simulink model "Sensor_Fusion_Simulink"  (R2025b)
settings: Solver=VariableStepAuto  StartTime=0.0  StopTime=30  RelTol=1e-3
undefined symbols (not defined in the file): DiscIntNeverNeededParam
libraries: simulink_extras x10, slpidlib x7, simulink x5
settings Model: Creator=Admin ROG  LastModifiedBy=Admin ROG

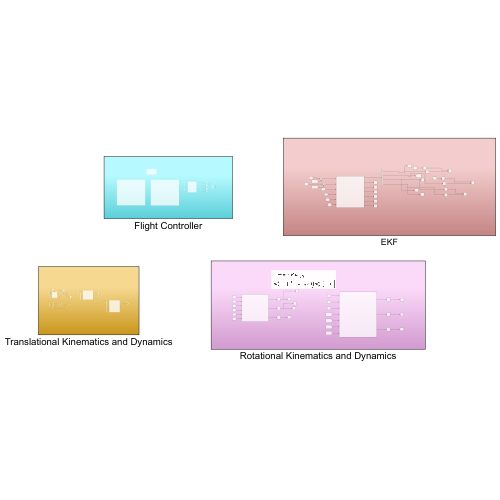
[thumbnail: Simulink's stored preview of the top-level diagram]
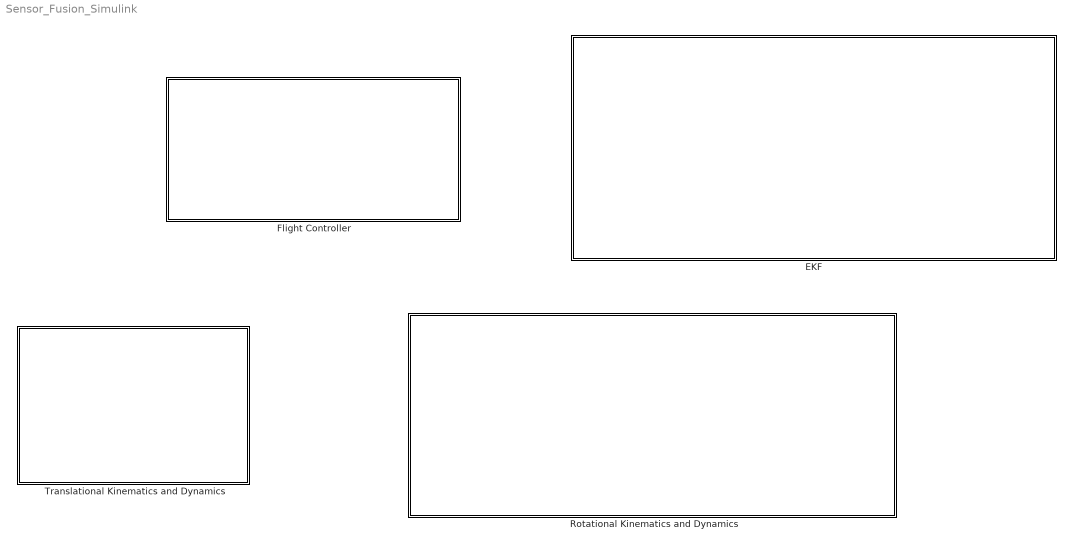
== system Sensor_Fusion_Simulink ==
  EKF : Subsystem
  Flight Controller : Subsystem
  Rotational Kinematics and Dynamics : Subsystem
  Translational Kinematics and Dynamics : Subsystem

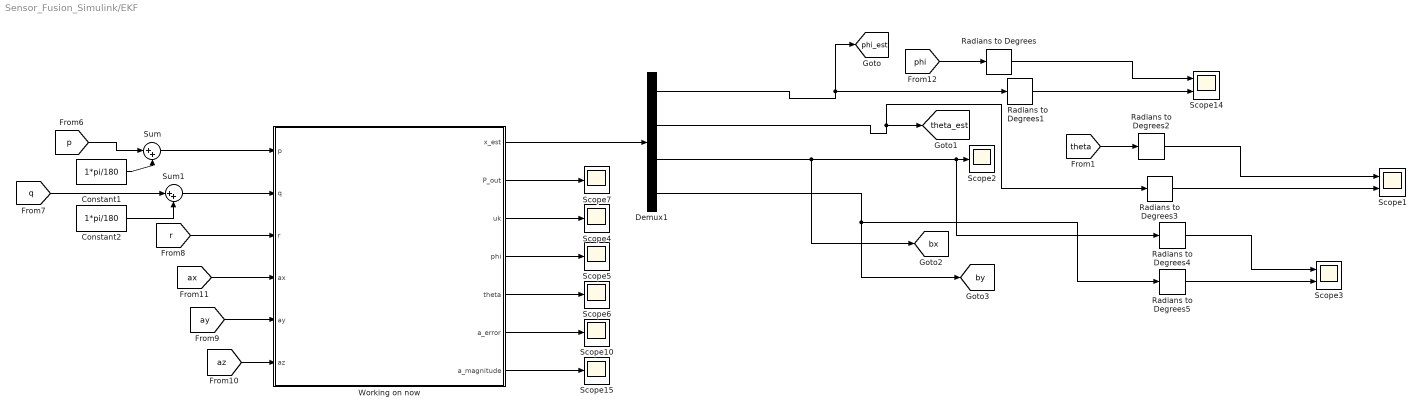
== system Sensor_Fusion_Simulink/EKF ==
  Constant1 : Constant  Value=1*pi/180
  Constant2 : Constant  Value=1*pi/180
  Demux1 : Demux
  Radians to Degrees{,1..5} (6 alike) : simulink_extras/Transformations/Radians to Degrees
  Scope1 : Scope  NumInputPorts=2
      settings: ActiveDisplayYMinimum=-0.57990177915773911  ActiveDisplayYMaximum=0.85703606877575134  DataLoggingVariableName=ScopeData19
  Scope{2,4..7,10,15} (7 alike) : Scope
      Scope10 settings: ActiveDisplayYMinimum=-33.495641453039809  ActiveDisplayYMaximum=182.18044745290689  DataLoggingVariableName=ScopeData35
      Scope15 settings: ActiveDisplayYMinimum=-33.295659158076418  ActiveDisplayYMaximum=317.12667362775773  DataLoggingVariableName=ScopeData36
      Scope2 settings: ActiveDisplayYMinimum=-0.0058388321761880082  ActiveDisplayYMaximum=0.025479521819259585  DataLoggingVariableName=ScopeData20
      Scope4 settings: ActiveDisplayYMinimum=-0.41125597879318471  ActiveDisplayYMaximum=3.5363536127434574  DataLoggingVariableName=ScopeData22
      Scope5 settings: ActiveDisplayYMinimum=-115.87931452635893  ActiveDisplayYMaximum=917.93819898150412  DataLoggingVariableName=ScopeData23
      Scope6 settings: ActiveDisplayYMinimum=-0.0043204427587799  ActiveDisplayYMaximum=0.014186886760105504  DataLoggingVariableName=ScopeData24
      Scope7 settings: ActiveDisplayYMinimum=-4.3708616172804561E-5  ActiveDisplayYMaximum=0.00012450012296327597  DataLoggingVariableName=ScopeData25
  Scope14 : Scope  NumInputPorts=2
      settings: ActiveDisplayYMinimum=-4.8648496704127089  ActiveDisplayYMaximum=36.951521266621747  DataLoggingVariableName=ScopeData18
  Scope3 : Scope  NumInputPorts=2
      settings: ActiveDisplayYMinimum=-0.33454044098075875  ActiveDisplayYMaximum=1.4598690642550676  DataLoggingVariableName=ScopeData21
  Sum : Sum  Inputs=|++
  Sum1 : Sum  Inputs=|++
  Working on now : MATLAB Function  TreatAsAtomicUnit=on
  tag scope: bx=global, by=global, phi_est=global, theta_est=global
  wires:
  Demux1/3 -> [bx], Radians to Degrees4/1, Scope2/1
  Sum/1 -> Working on now/1(p)
  Demux1/1 -> [phi_est], Radians to Degrees1/1
  [az] -> Working on now/6(az)
  [ax] -> Working on now/4(ax)
  [p] -> Sum/1
  Working on now/5(theta) -> Scope6/1
  Working on now/6(a_error) -> Scope10/1
  Demux1/4 -> [by], Radians to Degrees5/1
  Working on now/7(a_magnitude) -> Scope15/1
  Working on now/4(phi) -> Scope5/1
  [ay] -> Working on now/5(ay)
  Working on now/3(uk) -> Scope4/1
  Demux1/2 -> [theta_est], Radians to Degrees3/1
  Working on now/1(x_est) -> Demux1/1
  Working on now/2(P_out) -> Scope7/1
  [r] -> Working on now/3(r)
  [phi] -> Radians to Degrees/1
  Radians to Degrees/1 -> Scope14/1
  Radians to Degrees1/1 -> Scope14/2
  Constant1/1 -> Sum/2
  [q] -> Sum1/1
  Sum1/1 -> Working on now/2(q)
  Constant2/1 -> Sum1/2
  [theta] -> Radians to Degrees2/1
  Radians to Degrees2/1 -> Scope1/1
  Radians to Degrees3/1 -> Scope1/2
  Radians to Degrees4/1 -> Scope3/1
  Radians to Degrees5/1 -> Scope3/2

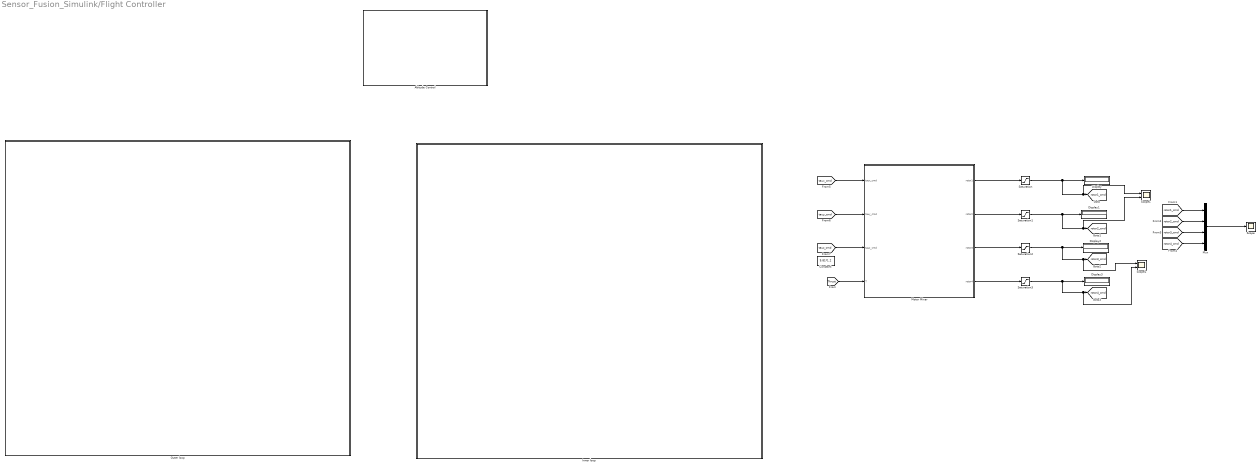
== system Sensor_Fusion_Simulink/Flight Controller ==
  Altitude Control : Subsystem
  Constant : Constant  Value=9.81*1.2
  Display{,1..3} (4 alike) : Display
  Inner loop : Subsystem
  Motor Mixer : MATLAB Function  TreatAsAtomicUnit=on
  Mux : Mux
  Outer loop : Subsystem
  Saturation{,1..3} (4 alike) : Saturate  UpperLimit=2094.8  LowerLimit=0
  Scope : Scope
      settings: ActiveDisplayYMinimum=-261.84999999999997  ActiveDisplayYMaximum=2356.65  DataLoggingVariableName=ScopeData7
  Scope1 : Scope  NumInputPorts=2
      settings: ActiveDisplayYMinimum=-261.84999999999997  ActiveDisplayYMaximum=2356.65  DataLoggingVariableName=ScopeData11
  Scope2 : Scope  NumInputPorts=2
      settings: ActiveDisplayYMinimum=820.27707495183745  ActiveDisplayYMaximum=820.27707495183768  DataLoggingVariableName=ScopeData12
  tag scope: rotor1_cmd=global, rotor2_cmd=global, rotor3_cmd=global, rotor4_cmd=global
  wires:
  [rotor2_cmd] -> Mux/2
  [rotor3_cmd] -> Mux/3
  Mux/1 -> Scope/1
  [rotor1_cmd] -> Mux/1
  [rotor4_cmd] -> Mux/4
  Motor Mixer/4(rotor4) -> Saturation3/1
  Motor Mixer/3(rotor3) -> Saturation2/1
  Motor Mixer/1(rotor1) -> Saturation/1
  Motor Mixer/2(rotor2) -> Saturation1/1
  Saturation/1 -> Scope1/1, [rotor1_cmd], Display/1
  Saturation1/1 -> Scope1/2, [rotor2_cmd], Display1/1
  Saturation2/1 -> Scope2/1, [rotor3_cmd], Display2/1
  Saturation3/1 -> Scope2/2, [rotor4_cmd], Display3/1
  [tauy_cmd] -> Motor Mixer/2(tauy_cmd)
  [taux_cmd] -> Motor Mixer/1(taux_cmd)
  [tauz_cmd] -> Motor Mixer/3(tauz_cmd)
  [Thrust] -> Motor Mixer/4(T)

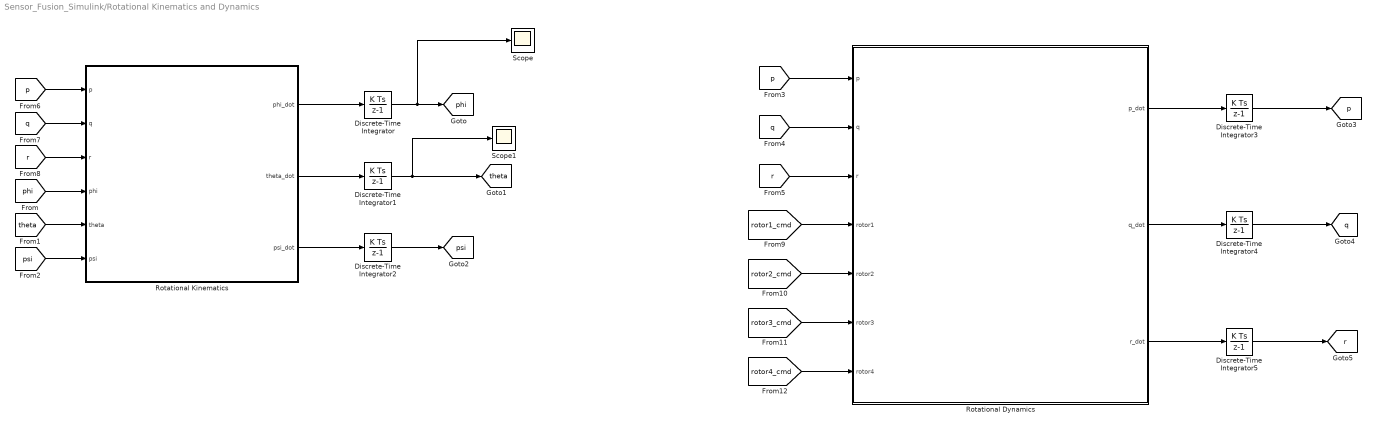
== system Sensor_Fusion_Simulink/Rotational Kinematics and Dynamics ==
  Discrete-Time Integrator{,1..5} (6 alike) : DiscreteIntegrator  SampleTime=0.002  ICPrevOutput=DiscIntNeverNeededParam  ICPrevScaledInput=DiscIntNeverNeededParam
  Rotational Dynamics : MATLAB Function  TreatAsAtomicUnit=on
  "Rotational Kinematics    " : MATLAB Function  TreatAsAtomicUnit=on
  Scope : Scope
      settings: ActiveDisplayYMinimum=-0.022412150722965766  ActiveDisplayYMaximum=0.028745169300771516  DataLoggingVariableName=ScopeData3
  Scope1 : Scope
      settings: ActiveDisplayYMinimum=-13.839906623900923  ActiveDisplayYMaximum=45.902212590490322  DataLoggingVariableName=ScopeData4
  tag scope: p=global, phi=global, psi=global, q=global, r=global, theta=global
  wires:
  Discrete-Time Integrator2/1 -> [psi]
  Discrete-Time Integrator4/1 -> [q]
  Discrete-Time Integrator/1 -> Scope/1, [phi]
  [psi] -> "Rotational Kinematics    "/6(psi)
  [theta] -> "Rotational Kinematics    "/5(theta)
  Discrete-Time Integrator3/1 -> [p]
  "Rotational Kinematics    "/1(phi_dot) -> Discrete-Time Integrator/1
  "Rotational Kinematics    "/2(theta_dot) -> Discrete-Time Integrator1/1
  "Rotational Kinematics    "/3(psi_dot) -> Discrete-Time Integrator2/1
  [phi] -> "Rotational Kinematics    "/4(phi)
  Rotational Dynamics/2(q_dot) -> Discrete-Time Integrator4/1
  Discrete-Time Integrator5/1 -> [r]
  Rotational Dynamics/3(r_dot) -> Discrete-Time Integrator5/1
  Rotational Dynamics/1(p_dot) -> Discrete-Time Integrator3/1
  [r] -> Rotational Dynamics/3(r)
  [q] -> Rotational Dynamics/2(q)
  [p] -> Rotational Dynamics/1(p)
  [p] -> "Rotational Kinematics    "/1(p)
  [q] -> "Rotational Kinematics    "/2(q)
  [r] -> "Rotational Kinematics    "/3(r)
  Discrete-Time Integrator1/1 -> Scope1/1, [theta]
  [rotor2_cmd] -> Rotational Dynamics/5(rotor2)
  [rotor1_cmd] -> Rotational Dynamics/4(rotor1)
  [rotor4_cmd] -> Rotational Dynamics/7(rotor4)
  [rotor3_cmd] -> Rotational Dynamics/6(rotor3)

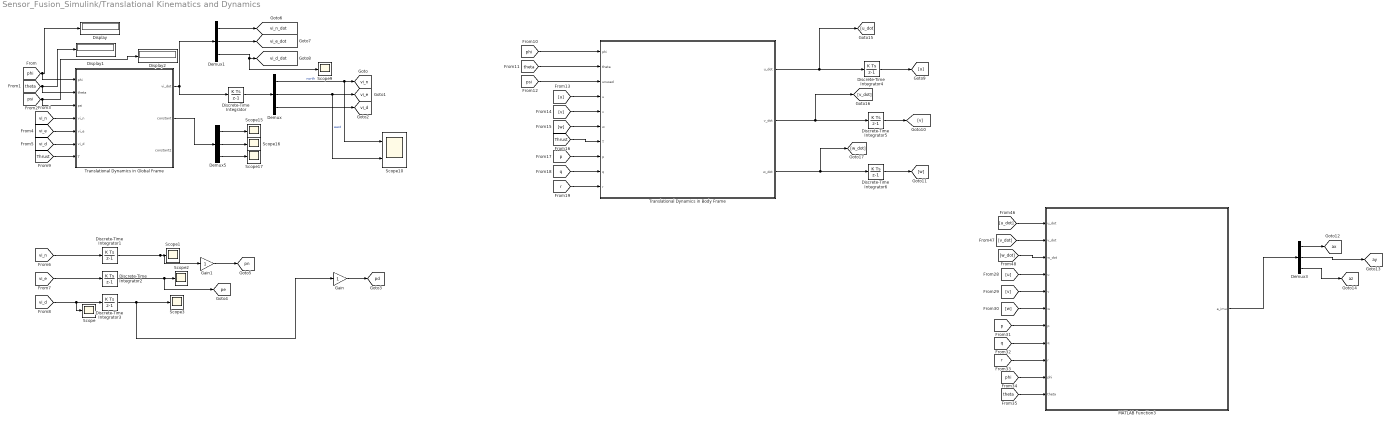
== system Sensor_Fusion_Simulink/Translational Kinematics and Dynamics ==
  Demux{,1,3,5} (4 alike) : Demux  Outputs=3
  Discrete-Time Integrator{,1..6} (7 alike) : DiscreteIntegrator  SampleTime=0.002  ICPrevOutput=DiscIntNeverNeededParam  ICPrevScaledInput=DiscIntNeverNeededParam
  Display : Display
  Display1 : Display
  Display2 : Display
  Gain : Gain
  Gain1 : Gain
  MATLAB Function3 : MATLAB Function  TreatAsAtomicUnit=on
  Scope{,1..3,9,15..17} (8 alike) : Scope
      Scope settings: ActiveDisplayYMinimum=-27.389318358760356  ActiveDisplayYMaximum=3.075052777222103  DataLoggingVariableName=ScopeData13
      Scope1 settings: ActiveDisplayYMinimum=-5.8001444763548868E-12  ActiveDisplayYMaximum=6.4446050675952019E-13
      Scope15 settings: ActiveDisplayYMinimum=-1.8377823013380582E-11  ActiveDisplayYMaximum=2.0419803348200644E-12  DataLoggingVariableName=ScopeData44
      Scope16 settings: ActiveDisplayYMinimum=-1  ActiveDisplayYMaximum=1  DataLoggingVariableName=ScopeData45
      Scope17 settings: ActiveDisplayYMinimum=0.91912060916271887  ActiveDisplayYMaximum=0.91912060917132532  DataLoggingVariableName=ScopeData46
      Scope2 settings: ActiveDisplayYMinimum=-5.2228944483105222  ActiveDisplayYMaximum=47.006050034794711
      Scope3 settings: ActiveDisplayYMinimum=-4898.5269794844062  ActiveDisplayYMaximum=544.28077549826719  DataLoggingVariableName=ScopeData2
      Scope9 settings: ActiveDisplayYMinimum=-247.424843275899  ActiveDisplayYMaximum=33.256922816424307  DataLoggingVariableName=ScopeData38
  Scope10 : Scope  NumInputPorts=2
      settings: ActiveDisplayYMinimum=-2.2562488531293E-16  ActiveDisplayYMaximum=6.7654414881576984E-17  DataLoggingVariableName=ScopeData39
  Translational Dynamics in Body Frame : MATLAB Function  TreatAsAtomicUnit=on
  Translational Dynamics in Global Frame : MATLAB Function  TreatAsAtomicUnit=on
  tag scope: ax=global, ay=global, az=global, pd=global, pe=global, pn=global, vi_d=global, vi_d_dot=global, vi_e=global, vi_e_dot=global, vi_n=global, vi_n_dot=global
  wires:
  [phi] -> Display/1, Translational Dynamics in Global Frame/1(phi)
  [theta] -> Display1/1, Translational Dynamics in Global Frame/2(theta)
  [psi] -> Display2/1, Translational Dynamics in Global Frame/3(psi)
  Translational Dynamics in Global Frame/1(vi_dot) -> Discrete-Time Integrator/1, Demux1/1
  Demux/1 -> Scope10/1, [vi_n]  "north"
  Demux/2 -> Scope10/2, [vi_e]  "east"
  Demux/3 -> [vi_d]
  [vi_n] -> Translational Dynamics in Global Frame/4(vi_n)
  [vi_e] -> Translational Dynamics in Global Frame/5(vi_e)
  [vi_d] -> Translational Dynamics in Global Frame/6(vi_d)
  Discrete-Time Integrator/1 -> Demux/1
  [vi_n] -> Discrete-Time Integrator1/1
  [vi_d] -> Scope/1, Discrete-Time Integrator3/1
  [vi_e] -> Discrete-Time Integrator2/1
  Discrete-Time Integrator1/1 -> Gain1/1, Scope1/1
  Discrete-Time Integrator2/1 -> Scope2/1, [pe]
  Discrete-Time Integrator3/1 -> Scope3/1, Gain/1
  Gain/1 -> [pd]
  Gain1/1 -> [pn]
  Demux1/1 -> [vi_n_dot]
  Demux1/2 -> [vi_e_dot]
  Demux1/3 -> Scope9/1, [vi_d_dot]
  [phi] -> Translational Dynamics in Body Frame/1(phi)
  [theta] -> Translational Dynamics in Body Frame/2(theta)
  [psi] -> Translational Dynamics in Body Frame/3(unused)
  Translational Dynamics in Body Frame/1(u_dot) -> [u_dot], Discrete-Time Integrator4/1
  Translational Dynamics in Body Frame/2(v_dot) -> [v_dot], Discrete-Time Integrator5/1
  Translational Dynamics in Body Frame/3(w_dot) -> [w_dot], Discrete-Time Integrator6/1
  [u] -> Translational Dynamics in Body Frame/4(u)
  [v] -> Translational Dynamics in Body Frame/5(v)
  [w] -> Translational Dynamics in Body Frame/6(w)
  [p] -> Translational Dynamics in Body Frame/8(p)
  [q] -> Translational Dynamics in Body Frame/9(q)
  [r] -> Translational Dynamics in Body Frame/10(r)
  [u] -> MATLAB Function3/4(u)
  [v] -> MATLAB Function3/5(v)
  [w] -> MATLAB Function3/6(w)
  [p] -> MATLAB Function3/7(p)
  [q] -> MATLAB Function3/8(q)
  [r] -> MATLAB Function3/9(r)
  [phi] -> MATLAB Function3/10(phi)
  [theta] -> MATLAB Function3/11(theta)
  MATLAB Function3/1(a_imu) -> Demux3/1
  Discrete-Time Integrator4/1 -> [u]
  Discrete-Time Integrator6/1 -> [w]
  Discrete-Time Integrator5/1 -> [v]
  Demux5/1 -> Scope15/1
  Demux5/2 -> Scope16/1
  Demux5/3 -> Scope17/1
  Translational Dynamics in Global Frame/2(constant) -> Demux5/1
  [w_dot] -> MATLAB Function3/3(w_dot)
  [u_dot] -> MATLAB Function3/1(u_dot)
  [v_dot] -> MATLAB Function3/2(v_dot)
  Demux3/1 -> [ax]
  Demux3/2 -> [ay]
  Demux3/3 -> [az]
  [Thrust] -> Translational Dynamics in Global Frame/7(T)
  [Thrust] -> Translational Dynamics in Body Frame/7(T)

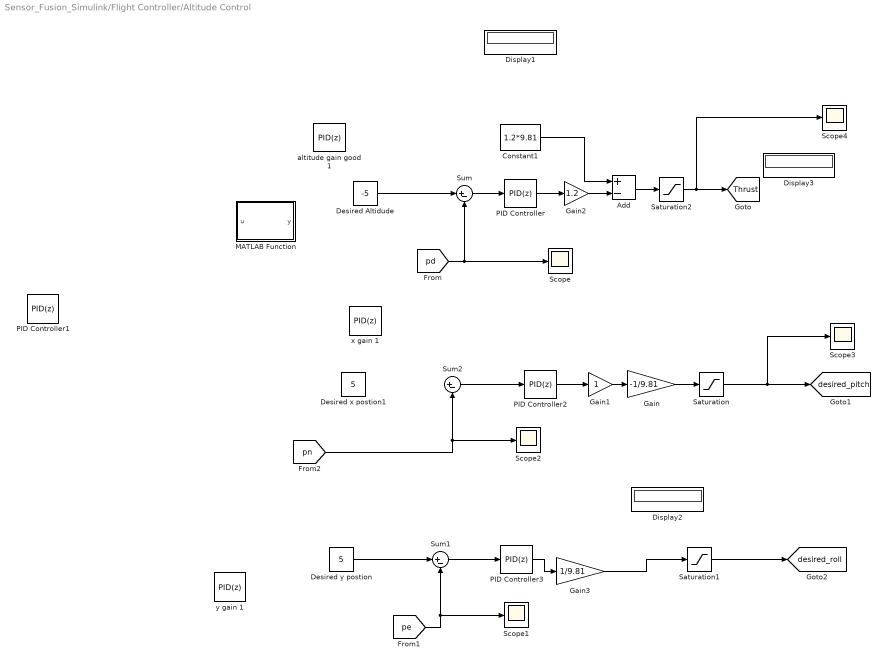
== system Sensor_Fusion_Simulink/Flight Controller/Altitude Control ==
  Add : Sum  Inputs=+-
  Constant1 : Constant  Value=1.2*9.81
  "Desired Altidude " : Constant  Value=-5
  Desired x postion1 : Constant  Value=5
  Desired y postion : Constant  Value=5
  Display1 : Display
  Display2 : Display
  Display3 : Display
  Gain : Gain  Gain=-1/9.81
  Gain1 : Gain
  Gain2 : Gain  Gain=1.2
  Gain3 : Gain  Gain=1/9.81
  MATLAB Function : MATLAB Function  TreatAsAtomicUnit=on
  PID Controller : slpidlib/PID Controller  Controller=PID  Form=Parallel  TimeDomain=Discrete-time  UseExternalTs=off  SampleTime=0.002  IntegratorMethod=Forward Euler  FilterMethod=Forward Euler  ControllerParametersSource=internal  P=3  I=0  UseKiTs=off  D=3  UseExternalDerivativeSource=off  N=100  UseFilter=on  TunerSelectOption=Transfer Function Based (PID Tuner App)  InitialConditionSource=internal  InitialConditionForIntegrator=0  InitialConditionForFilter=0  DifferentiatorICPrevScaledInput=0  ExternalReset=none  TrackingMode=off  Kt=1  LimitOutput=off  SatLimitsSource=internal  UpperSaturationLimit=inf  LowerSaturationLimit=-inf  LinearizeAsGain=on  AntiWindupMode=none  Kb=1  LimitIntegrator=off  UpperIntegratorSaturationLimit=inf  LowerIntegratorSaturationLimit=-inf  POutMin=[]  POutMax=[]  IOutMin=[]  IOutMax=[]  DOutMin=[]  DOutMax=[]  NOutMin=[]  NOutMax=[]  SumOutMin=[]  SumOutMax=[]  SaturationOutMin=[]  SaturationOutMax=[]  PParamMin=[]  PParamMax=[]  IParamMin=[]  IParamMax=[]  DParamMin=[]  DParamMax=[]  NParamMin=[]  NParamMax=[]  KbParamMin=[]  KbParamMax=[]  KtParamMin=[]  KtParamMax=[]  KbOutMin=[]  KbOutMax=[]  KtOutMin=[]  KtOutMax=[]  IntegratorOutMin=[]  IntegratorOutMax=[]  FilterOutMin=[]  FilterOutMax=[]  SumI1OutMin=[]  SumI1OutMax=[]  SumI2OutMin=[]  SumI2OutMax=[]  SumI3OutMin=[]  SumI3OutMax=[]  SumI4OutMin=[]  SumI4OutMax=[]  SumDOutMin=[]  SumDOutMax=[]  DifferentiatorOutMin=[]  DifferentiatorOutMax=[]  FilterDiffOutCoefMin=[]  FilterDiffOutCoefMax=[]  ReciprocalOutMin=[]  ReciprocalOutMax=[]  SumDenOutMin=[]  SumDenOutMax=[]  SumNumOutMin=[]  SumNumOutMax=[]  DivideOutMin=[]  DivideOutMax=[]  UdiffTsProdOutMin=[]  UdiffTsProdOutMax=[]  NTsProdOutMin=[]  NTsProdOutMax=[]  UintegralTsProdOutMin=[]  UintegralTsProdOutMax=[]  UngainTsProdOutMin=[]  UngainTsProdOutMax=[]  ClampingZeroOutDataTypeStr=Inherit: Inherit via back propagation  ClampingZeroOutMin=[]  ClampingZeroOutMax=[]  FilterDenConstantOutDataTypeStr=Inherit: Inherit via back propagation  FilterDenConstantOutMin=[]  FilterDenConstantOutMax=[]  PCopyOutDataTypeStr=Inherit: Inherit via back propagation  PCopyOutMin=[]  PCopyOutMax=[]  NCopyOutDataTypeStr=Inherit: Inherit via back propagation  NCopyOutMin=[]  NCopyOutMax=[]  IntegratorContinuousStateAttributes=''  IntegratorStateMustResolveToSignalObject=off  IntegratorRTWStateStorageClass=Auto  FilterContinuousStateAttributes=''  FilterStateMustResolveToSignalObject=off  FilterRTWStateStorageClass=Auto  ParallelPVariant=InternalParameters  IdealPVariant=Disabled  IVariant=InternalParameters  DVariant=InternalParameters  IntegratorVariant=Discrete  SatVariant=Disabled  AWVariant=Passthrough  PCopyVariant=Disabled  TRVariant=Disabled  FdbkBlocksVariant=Forward  IdealPFdbkVariant=Disabled  SatFdbkVariant=Disabled  DerivativeFilterVariant=ForwardEulerFilter  NVariant=InternalParameters  NCopyVariant=Disabled  FilterICVariant=InternalICsFilter  IntegratorICVariant=InternalICs  ExternalResetVariant=Disabled  TRSumVariant=Passthrough  SumFdbkVariant=Disabled  SumVariant=Sum_PID  TsampFilterVariant=InternalTs  TsampNgainVariant=Passthrough  TsampIntegralVariant=Disabled_SignalSpec  ExternalSaturationOutDataTypeStr=Inherit: Same as second input  DerivativeSourceVariant=ErrorSignal  PreIntVariant=InternalPreInt
  PID Controller1 : slpidlib/PID Controller  Controller=PID  Form=Parallel  TimeDomain=Discrete-time  UseExternalTs=off  SampleTime=0.02  IntegratorMethod=Forward Euler  FilterMethod=Forward Euler  ControllerParametersSource=internal  P=0.5  I=0  UseKiTs=off  D=1  UseExternalDerivativeSource=off  N=20  UseFilter=on  TunerSelectOption=Transfer Function Based (PID Tuner App)  InitialConditionSource=internal  InitialConditionForIntegrator=0  InitialConditionForFilter=0  DifferentiatorICPrevScaledInput=0  ExternalReset=none  TrackingMode=off  Kt=1  LimitOutput=off  SatLimitsSource=internal  UpperSaturationLimit=inf  LowerSaturationLimit=-inf  LinearizeAsGain=on  AntiWindupMode=none  Kb=1  LimitIntegrator=off  UpperIntegratorSaturationLimit=inf  LowerIntegratorSaturationLimit=-inf  POutMin=[]  POutMax=[]  IOutMin=[]  IOutMax=[]  DOutMin=[]  DOutMax=[]  NOutMin=[]  NOutMax=[]  SumOutMin=[]  SumOutMax=[]  SaturationOutMin=[]  SaturationOutMax=[]  PParamMin=[]  PParamMax=[]  IParamMin=[]  IParamMax=[]  DParamMin=[]  DParamMax=[]  NParamMin=[]  NParamMax=[]  KbParamMin=[]  KbParamMax=[]  KtParamMin=[]  KtParamMax=[]  KbOutMin=[]  KbOutMax=[]  KtOutMin=[]  KtOutMax=[]  IntegratorOutMin=[]  IntegratorOutMax=[]  FilterOutMin=[]  FilterOutMax=[]  SumI1OutMin=[]  SumI1OutMax=[]  SumI2OutMin=[]  SumI2OutMax=[]  SumI3OutMin=[]  SumI3OutMax=[]  SumI4OutMin=[]  SumI4OutMax=[]  SumDOutMin=[]  SumDOutMax=[]  DifferentiatorOutMin=[]  DifferentiatorOutMax=[]  FilterDiffOutCoefMin=[]  FilterDiffOutCoefMax=[]  ReciprocalOutMin=[]  ReciprocalOutMax=[]  SumDenOutMin=[]  SumDenOutMax=[]  SumNumOutMin=[]  SumNumOutMax=[]  DivideOutMin=[]  DivideOutMax=[]  UdiffTsProdOutMin=[]  UdiffTsProdOutMax=[]  NTsProdOutMin=[]  NTsProdOutMax=[]  UintegralTsProdOutMin=[]  UintegralTsProdOutMax=[]  UngainTsProdOutMin=[]  UngainTsProdOutMax=[]  ClampingZeroOutDataTypeStr=Inherit: Inherit via back propagation  ClampingZeroOutMin=[]  ClampingZeroOutMax=[]  FilterDenConstantOutDataTypeStr=Inherit: Inherit via back propagation  FilterDenConstantOutMin=[]  FilterDenConstantOutMax=[]  PCopyOutDataTypeStr=Inherit: Inherit via back propagation  PCopyOutMin=[]  PCopyOutMax=[]  NCopyOutDataTypeStr=Inherit: Inherit via back propagation  NCopyOutMin=[]  NCopyOutMax=[]  IntegratorContinuousStateAttributes=''  IntegratorStateMustResolveToSignalObject=off  IntegratorRTWStateStorageClass=Auto  FilterContinuousStateAttributes=''  FilterStateMustResolveToSignalObject=off  FilterRTWStateStorageClass=Auto  ParallelPVariant=InternalParameters  IdealPVariant=Disabled  IVariant=InternalParameters  DVariant=InternalParameters  IntegratorVariant=Discrete  SatVariant=Disabled  AWVariant=Passthrough  PCopyVariant=Disabled  TRVariant=Disabled  FdbkBlocksVariant=Forward  IdealPFdbkVariant=Disabled  SatFdbkVariant=Disabled  DerivativeFilterVariant=ForwardEulerFilter  NVariant=InternalParameters  NCopyVariant=Disabled  FilterICVariant=InternalICsFilter  IntegratorICVariant=InternalICs  ExternalResetVariant=Disabled  TRSumVariant=Passthrough  SumFdbkVariant=Disabled  SumVariant=Sum_PID  TsampFilterVariant=InternalTs  TsampNgainVariant=Passthrough  TsampIntegralVariant=Disabled_SignalSpec  ExternalSaturationOutDataTypeStr=Inherit: Same as second input  DerivativeSourceVariant=ErrorSignal  PreIntVariant=InternalPreInt
  PID Controller2 : slpidlib/PID Controller  Controller=PID  Form=Parallel  TimeDomain=Discrete-time  UseExternalTs=off  SampleTime=0.02  IntegratorMethod=Forward Euler  FilterMethod=Forward Euler  ControllerParametersSource=internal  P=0.5  I=0  UseKiTs=off  D=2  UseExternalDerivativeSource=off  N=20  UseFilter=on  TunerSelectOption=Transfer Function Based (PID Tuner App)  InitialConditionSource=internal  InitialConditionForIntegrator=0  InitialConditionForFilter=0  DifferentiatorICPrevScaledInput=0  ExternalReset=none  TrackingMode=off  Kt=1  LimitOutput=off  SatLimitsSource=internal  UpperSaturationLimit=inf  LowerSaturationLimit=-inf  LinearizeAsGain=on  AntiWindupMode=none  Kb=1  LimitIntegrator=off  UpperIntegratorSaturationLimit=inf  LowerIntegratorSaturationLimit=-inf  POutMin=[]  POutMax=[]  IOutMin=[]  IOutMax=[]  DOutMin=[]  DOutMax=[]  NOutMin=[]  NOutMax=[]  SumOutMin=[]  SumOutMax=[]  SaturationOutMin=[]  SaturationOutMax=[]  PParamMin=[]  PParamMax=[]  IParamMin=[]  IParamMax=[]  DParamMin=[]  DParamMax=[]  NParamMin=[]  NParamMax=[]  KbParamMin=[]  KbParamMax=[]  KtParamMin=[]  KtParamMax=[]  KbOutMin=[]  KbOutMax=[]  KtOutMin=[]  KtOutMax=[]  IntegratorOutMin=[]  IntegratorOutMax=[]  FilterOutMin=[]  FilterOutMax=[]  SumI1OutMin=[]  SumI1OutMax=[]  SumI2OutMin=[]  SumI2OutMax=[]  SumI3OutMin=[]  SumI3OutMax=[]  SumI4OutMin=[]  SumI4OutMax=[]  SumDOutMin=[]  SumDOutMax=[]  DifferentiatorOutMin=[]  DifferentiatorOutMax=[]  FilterDiffOutCoefMin=[]  FilterDiffOutCoefMax=[]  ReciprocalOutMin=[]  ReciprocalOutMax=[]  SumDenOutMin=[]  SumDenOutMax=[]  SumNumOutMin=[]  SumNumOutMax=[]  DivideOutMin=[]  DivideOutMax=[]  UdiffTsProdOutMin=[]  UdiffTsProdOutMax=[]  NTsProdOutMin=[]  NTsProdOutMax=[]  UintegralTsProdOutMin=[]  UintegralTsProdOutMax=[]  UngainTsProdOutMin=[]  UngainTsProdOutMax=[]  ClampingZeroOutDataTypeStr=Inherit: Inherit via back propagation  ClampingZeroOutMin=[]  ClampingZeroOutMax=[]  FilterDenConstantOutDataTypeStr=Inherit: Inherit via back propagation  FilterDenConstantOutMin=[]  FilterDenConstantOutMax=[]  PCopyOutDataTypeStr=Inherit: Inherit via back propagation  PCopyOutMin=[]  PCopyOutMax=[]  NCopyOutDataTypeStr=Inherit: Inherit via back propagation  NCopyOutMin=[]  NCopyOutMax=[]  IntegratorContinuousStateAttributes=''  IntegratorStateMustResolveToSignalObject=off  IntegratorRTWStateStorageClass=Auto  FilterContinuousStateAttributes=''  FilterStateMustResolveToSignalObject=off  FilterRTWStateStorageClass=Auto  ParallelPVariant=InternalParameters  IdealPVariant=Disabled  IVariant=InternalParameters  DVariant=InternalParameters  IntegratorVariant=Discrete  SatVariant=Disabled  AWVariant=Passthrough  PCopyVariant=Disabled  TRVariant=Disabled  FdbkBlocksVariant=Forward  IdealPFdbkVariant=Disabled  SatFdbkVariant=Disabled  DerivativeFilterVariant=ForwardEulerFilter  NVariant=InternalParameters  NCopyVariant=Disabled  FilterICVariant=InternalICsFilter  IntegratorICVariant=InternalICs  ExternalResetVariant=Disabled  TRSumVariant=Passthrough  SumFdbkVariant=Disabled  SumVariant=Sum_PID  TsampFilterVariant=InternalTs  TsampNgainVariant=Passthrough  TsampIntegralVariant=Disabled_SignalSpec  ExternalSaturationOutDataTypeStr=Inherit: Same as second input  DerivativeSourceVariant=ErrorSignal  PreIntVariant=InternalPreInt
  PID Controller3 : slpidlib/PID Controller  Controller=PID  Form=Parallel  TimeDomain=Discrete-time  UseExternalTs=off  SampleTime=0.02  IntegratorMethod=Forward Euler  FilterMethod=Forward Euler  ControllerParametersSource=internal  P=0.5  I=0  UseKiTs=off  D=1.8  UseExternalDerivativeSource=off  N=20  UseFilter=on  TunerSelectOption=Transfer Function Based (PID Tuner App)  InitialConditionSource=internal  InitialConditionForIntegrator=0  InitialConditionForFilter=0  DifferentiatorICPrevScaledInput=0  ExternalReset=none  TrackingMode=off  Kt=1  LimitOutput=off  SatLimitsSource=internal  UpperSaturationLimit=inf  LowerSaturationLimit=-inf  LinearizeAsGain=on  AntiWindupMode=none  Kb=1  LimitIntegrator=off  UpperIntegratorSaturationLimit=inf  LowerIntegratorSaturationLimit=-inf  POutMin=[]  POutMax=[]  IOutMin=[]  IOutMax=[]  DOutMin=[]  DOutMax=[]  NOutMin=[]  NOutMax=[]  SumOutMin=[]  SumOutMax=[]  SaturationOutMin=[]  SaturationOutMax=[]  PParamMin=[]  PParamMax=[]  IParamMin=[]  IParamMax=[]  DParamMin=[]  DParamMax=[]  NParamMin=[]  NParamMax=[]  KbParamMin=[]  KbParamMax=[]  KtParamMin=[]  KtParamMax=[]  KbOutMin=[]  KbOutMax=[]  KtOutMin=[]  KtOutMax=[]  IntegratorOutMin=[]  IntegratorOutMax=[]  FilterOutMin=[]  FilterOutMax=[]  SumI1OutMin=[]  SumI1OutMax=[]  SumI2OutMin=[]  SumI2OutMax=[]  SumI3OutMin=[]  SumI3OutMax=[]  SumI4OutMin=[]  SumI4OutMax=[]  SumDOutMin=[]  SumDOutMax=[]  DifferentiatorOutMin=[]  DifferentiatorOutMax=[]  FilterDiffOutCoefMin=[]  FilterDiffOutCoefMax=[]  ReciprocalOutMin=[]  ReciprocalOutMax=[]  SumDenOutMin=[]  SumDenOutMax=[]  SumNumOutMin=[]  SumNumOutMax=[]  DivideOutMin=[]  DivideOutMax=[]  UdiffTsProdOutMin=[]  UdiffTsProdOutMax=[]  NTsProdOutMin=[]  NTsProdOutMax=[]  UintegralTsProdOutMin=[]  UintegralTsProdOutMax=[]  UngainTsProdOutMin=[]  UngainTsProdOutMax=[]  ClampingZeroOutDataTypeStr=Inherit: Inherit via back propagation  ClampingZeroOutMin=[]  ClampingZeroOutMax=[]  FilterDenConstantOutDataTypeStr=Inherit: Inherit via back propagation  FilterDenConstantOutMin=[]  FilterDenConstantOutMax=[]  PCopyOutDataTypeStr=Inherit: Inherit via back propagation  PCopyOutMin=[]  PCopyOutMax=[]  NCopyOutDataTypeStr=Inherit: Inherit via back propagation  NCopyOutMin=[]  NCopyOutMax=[]  IntegratorContinuousStateAttributes=''  IntegratorStateMustResolveToSignalObject=off  IntegratorRTWStateStorageClass=Auto  FilterContinuousStateAttributes=''  FilterStateMustResolveToSignalObject=off  FilterRTWStateStorageClass=Auto  ParallelPVariant=InternalParameters  IdealPVariant=Disabled  IVariant=InternalParameters  DVariant=InternalParameters  IntegratorVariant=Discrete  SatVariant=Disabled  AWVariant=Passthrough  PCopyVariant=Disabled  TRVariant=Disabled  FdbkBlocksVariant=Forward  IdealPFdbkVariant=Disabled  SatFdbkVariant=Disabled  DerivativeFilterVariant=ForwardEulerFilter  NVariant=InternalParameters  NCopyVariant=Disabled  FilterICVariant=InternalICsFilter  IntegratorICVariant=InternalICs  ExternalResetVariant=Disabled  TRSumVariant=Passthrough  SumFdbkVariant=Disabled  SumVariant=Sum_PID  TsampFilterVariant=InternalTs  TsampNgainVariant=Passthrough  TsampIntegralVariant=Disabled_SignalSpec  ExternalSaturationOutDataTypeStr=Inherit: Same as second input  DerivativeSourceVariant=ErrorSignal  PreIntVariant=InternalPreInt
  Saturation : Saturate  UpperLimit=45*pi/180  LowerLimit=-45*pi/180
  Saturation1 : Saturate  UpperLimit=45*pi/180  LowerLimit=-45*pi/180
  Saturation2 : Saturate  UpperLimit=275  LowerLimit=0
  Scope{,1..4} (5 alike) : Scope
      Scope settings: ActiveDisplayYMinimum=-5.6552923105133956  ActiveDisplayYMaximum=0.628365812279266  DataLoggingVariableName=ScopeData14
      Scope1 settings: ActiveDisplayYMinimum=-0.62598234186213919  ActiveDisplayYMaximum=5.6338410767592535  DataLoggingVariableName=ScopeData15
      Scope2 settings: ActiveDisplayYMinimum=-0.021314976158697256  ActiveDisplayYMaximum=0.18898032291094422  DataLoggingVariableName=ScopeData16
      Scope3 settings: ActiveDisplayYMinimum=-0.002897548084977811  ActiveDisplayYMaximum=0.015571132830339837  DataLoggingVariableName=ScopeData17
      Scope4 settings: ActiveDisplayYMinimum=-26.929946110527347  ActiveDisplayYMaximum=308.54777179005862  DataLoggingVariableName=ScopeData41
  Sum : Sum  Inputs=|+-
  Sum1 : Sum  Inputs=|+-
  Sum2 : Sum  Inputs=|+-
  altitude gain good 1 : slpidlib/PID Controller  Controller=PID  Form=Parallel  TimeDomain=Discrete-time  UseExternalTs=off  SampleTime=0.02  IntegratorMethod=Forward Euler  FilterMethod=Forward Euler  ControllerParametersSource=internal  P=4  I=0  UseKiTs=off  D=5  UseExternalDerivativeSource=off  N=100  UseFilter=on  TunerSelectOption=Transfer Function Based (PID Tuner App)  InitialConditionSource=internal  InitialConditionForIntegrator=0  InitialConditionForFilter=0  DifferentiatorICPrevScaledInput=0  ExternalReset=none  TrackingMode=off  Kt=1  LimitOutput=off  SatLimitsSource=internal  UpperSaturationLimit=inf  LowerSaturationLimit=-inf  LinearizeAsGain=on  AntiWindupMode=none  Kb=1  LimitIntegrator=off  UpperIntegratorSaturationLimit=inf  LowerIntegratorSaturationLimit=-inf  POutMin=[]  POutMax=[]  IOutMin=[]  IOutMax=[]  DOutMin=[]  DOutMax=[]  NOutMin=[]  NOutMax=[]  SumOutMin=[]  SumOutMax=[]  SaturationOutMin=[]  SaturationOutMax=[]  PParamMin=[]  PParamMax=[]  IParamMin=[]  IParamMax=[]  DParamMin=[]  DParamMax=[]  NParamMin=[]  NParamMax=[]  KbParamMin=[]  KbParamMax=[]  KtParamMin=[]  KtParamMax=[]  KbOutMin=[]  KbOutMax=[]  KtOutMin=[]  KtOutMax=[]  IntegratorOutMin=[]  IntegratorOutMax=[]  FilterOutMin=[]  FilterOutMax=[]  SumI1OutMin=[]  SumI1OutMax=[]  SumI2OutMin=[]  SumI2OutMax=[]  SumI3OutMin=[]  SumI3OutMax=[]  SumI4OutMin=[]  SumI4OutMax=[]  SumDOutMin=[]  SumDOutMax=[]  DifferentiatorOutMin=[]  DifferentiatorOutMax=[]  FilterDiffOutCoefMin=[]  FilterDiffOutCoefMax=[]  ReciprocalOutMin=[]  ReciprocalOutMax=[]  SumDenOutMin=[]  SumDenOutMax=[]  SumNumOutMin=[]  SumNumOutMax=[]  DivideOutMin=[]  DivideOutMax=[]  UdiffTsProdOutMin=[]  UdiffTsProdOutMax=[]  NTsProdOutMin=[]  NTsProdOutMax=[]  UintegralTsProdOutMin=[]  UintegralTsProdOutMax=[]  UngainTsProdOutMin=[]  UngainTsProdOutMax=[]  ClampingZeroOutDataTypeStr=Inherit: Inherit via back propagation  ClampingZeroOutMin=[]  ClampingZeroOutMax=[]  FilterDenConstantOutDataTypeStr=Inherit: Inherit via back propagation  FilterDenConstantOutMin=[]  FilterDenConstantOutMax=[]  PCopyOutDataTypeStr=Inherit: Inherit via back propagation  PCopyOutMin=[]  PCopyOutMax=[]  NCopyOutDataTypeStr=Inherit: Inherit via back propagation  NCopyOutMin=[]  NCopyOutMax=[]  IntegratorContinuousStateAttributes=''  IntegratorStateMustResolveToSignalObject=off  IntegratorRTWStateStorageClass=Auto  FilterContinuousStateAttributes=''  FilterStateMustResolveToSignalObject=off  FilterRTWStateStorageClass=Auto  ParallelPVariant=InternalParameters  IdealPVariant=Disabled  IVariant=InternalParameters  DVariant=InternalParameters  IntegratorVariant=Discrete  SatVariant=Disabled  AWVariant=Passthrough  PCopyVariant=Disabled  TRVariant=Disabled  FdbkBlocksVariant=Forward  IdealPFdbkVariant=Disabled  SatFdbkVariant=Disabled  DerivativeFilterVariant=ForwardEulerFilter  NVariant=InternalParameters  NCopyVariant=Disabled  FilterICVariant=InternalICsFilter  IntegratorICVariant=InternalICs  ExternalResetVariant=Disabled  TRSumVariant=Passthrough  SumFdbkVariant=Disabled  SumVariant=Sum_PID  TsampFilterVariant=InternalTs  TsampNgainVariant=Passthrough  TsampIntegralVariant=Disabled_SignalSpec  ExternalSaturationOutDataTypeStr=Inherit: Same as second input  DerivativeSourceVariant=ErrorSignal  PreIntVariant=InternalPreInt
  x gain 1 : slpidlib/PID Controller  Controller=PID  Form=Parallel  TimeDomain=Discrete-time  UseExternalTs=off  SampleTime=0.02  IntegratorMethod=Forward Euler  FilterMethod=Forward Euler  ControllerParametersSource=internal  P=0.3  I=0  UseKiTs=off  D=0.65  UseExternalDerivativeSource=off  N=20  UseFilter=on  TunerSelectOption=Transfer Function Based (PID Tuner App)  InitialConditionSource=internal  InitialConditionForIntegrator=0  InitialConditionForFilter=0  DifferentiatorICPrevScaledInput=0  ExternalReset=none  TrackingMode=off  Kt=1  LimitOutput=off  SatLimitsSource=internal  UpperSaturationLimit=inf  LowerSaturationLimit=-inf  LinearizeAsGain=on  AntiWindupMode=none  Kb=1  LimitIntegrator=off  UpperIntegratorSaturationLimit=inf  LowerIntegratorSaturationLimit=-inf  POutMin=[]  POutMax=[]  IOutMin=[]  IOutMax=[]  DOutMin=[]  DOutMax=[]  NOutMin=[]  NOutMax=[]  SumOutMin=[]  SumOutMax=[]  SaturationOutMin=[]  SaturationOutMax=[]  PParamMin=[]  PParamMax=[]  IParamMin=[]  IParamMax=[]  DParamMin=[]  DParamMax=[]  NParamMin=[]  NParamMax=[]  KbParamMin=[]  KbParamMax=[]  KtParamMin=[]  KtParamMax=[]  KbOutMin=[]  KbOutMax=[]  KtOutMin=[]  KtOutMax=[]  IntegratorOutMin=[]  IntegratorOutMax=[]  FilterOutMin=[]  FilterOutMax=[]  SumI1OutMin=[]  SumI1OutMax=[]  SumI2OutMin=[]  SumI2OutMax=[]  SumI3OutMin=[]  SumI3OutMax=[]  SumI4OutMin=[]  SumI4OutMax=[]  SumDOutMin=[]  SumDOutMax=[]  DifferentiatorOutMin=[]  DifferentiatorOutMax=[]  FilterDiffOutCoefMin=[]  FilterDiffOutCoefMax=[]  ReciprocalOutMin=[]  ReciprocalOutMax=[]  SumDenOutMin=[]  SumDenOutMax=[]  SumNumOutMin=[]  SumNumOutMax=[]  DivideOutMin=[]  DivideOutMax=[]  UdiffTsProdOutMin=[]  UdiffTsProdOutMax=[]  NTsProdOutMin=[]  NTsProdOutMax=[]  UintegralTsProdOutMin=[]  UintegralTsProdOutMax=[]  UngainTsProdOutMin=[]  UngainTsProdOutMax=[]  ClampingZeroOutDataTypeStr=Inherit: Inherit via back propagation  ClampingZeroOutMin=[]  ClampingZeroOutMax=[]  FilterDenConstantOutDataTypeStr=Inherit: Inherit via back propagation  FilterDenConstantOutMin=[]  FilterDenConstantOutMax=[]  PCopyOutDataTypeStr=Inherit: Inherit via back propagation  PCopyOutMin=[]  PCopyOutMax=[]  NCopyOutDataTypeStr=Inherit: Inherit via back propagation  NCopyOutMin=[]  NCopyOutMax=[]  IntegratorContinuousStateAttributes=''  IntegratorStateMustResolveToSignalObject=off  IntegratorRTWStateStorageClass=Auto  FilterContinuousStateAttributes=''  FilterStateMustResolveToSignalObject=off  FilterRTWStateStorageClass=Auto  ParallelPVariant=InternalParameters  IdealPVariant=Disabled  IVariant=InternalParameters  DVariant=InternalParameters  IntegratorVariant=Discrete  SatVariant=Disabled  AWVariant=Passthrough  PCopyVariant=Disabled  TRVariant=Disabled  FdbkBlocksVariant=Forward  IdealPFdbkVariant=Disabled  SatFdbkVariant=Disabled  DerivativeFilterVariant=ForwardEulerFilter  NVariant=InternalParameters  NCopyVariant=Disabled  FilterICVariant=InternalICsFilter  IntegratorICVariant=InternalICs  ExternalResetVariant=Disabled  TRSumVariant=Passthrough  SumFdbkVariant=Disabled  SumVariant=Sum_PID  TsampFilterVariant=InternalTs  TsampNgainVariant=Passthrough  TsampIntegralVariant=Disabled_SignalSpec  ExternalSaturationOutDataTypeStr=Inherit: Same as second input  DerivativeSourceVariant=ErrorSignal  PreIntVariant=InternalPreInt
  y gain 1 : slpidlib/PID Controller  Controller=PID  Form=Parallel  TimeDomain=Discrete-time  UseExternalTs=off  SampleTime=0.02  IntegratorMethod=Forward Euler  FilterMethod=Forward Euler  ControllerParametersSource=internal  P=0.6  I=0  UseKiTs=off  D=0.7  UseExternalDerivativeSource=off  N=20  UseFilter=on  TunerSelectOption=Transfer Function Based (PID Tuner App)  InitialConditionSource=internal  InitialConditionForIntegrator=0  InitialConditionForFilter=0  DifferentiatorICPrevScaledInput=0  ExternalReset=none  TrackingMode=off  Kt=1  LimitOutput=off  SatLimitsSource=internal  UpperSaturationLimit=inf  LowerSaturationLimit=-inf  LinearizeAsGain=on  AntiWindupMode=none  Kb=1  LimitIntegrator=off  UpperIntegratorSaturationLimit=inf  LowerIntegratorSaturationLimit=-inf  POutMin=[]  POutMax=[]  IOutMin=[]  IOutMax=[]  DOutMin=[]  DOutMax=[]  NOutMin=[]  NOutMax=[]  SumOutMin=[]  SumOutMax=[]  SaturationOutMin=[]  SaturationOutMax=[]  PParamMin=[]  PParamMax=[]  IParamMin=[]  IParamMax=[]  DParamMin=[]  DParamMax=[]  NParamMin=[]  NParamMax=[]  KbParamMin=[]  KbParamMax=[]  KtParamMin=[]  KtParamMax=[]  KbOutMin=[]  KbOutMax=[]  KtOutMin=[]  KtOutMax=[]  IntegratorOutMin=[]  IntegratorOutMax=[]  FilterOutMin=[]  FilterOutMax=[]  SumI1OutMin=[]  SumI1OutMax=[]  SumI2OutMin=[]  SumI2OutMax=[]  SumI3OutMin=[]  SumI3OutMax=[]  SumI4OutMin=[]  SumI4OutMax=[]  SumDOutMin=[]  SumDOutMax=[]  DifferentiatorOutMin=[]  DifferentiatorOutMax=[]  FilterDiffOutCoefMin=[]  FilterDiffOutCoefMax=[]  ReciprocalOutMin=[]  ReciprocalOutMax=[]  SumDenOutMin=[]  SumDenOutMax=[]  SumNumOutMin=[]  SumNumOutMax=[]  DivideOutMin=[]  DivideOutMax=[]  UdiffTsProdOutMin=[]  UdiffTsProdOutMax=[]  NTsProdOutMin=[]  NTsProdOutMax=[]  UintegralTsProdOutMin=[]  UintegralTsProdOutMax=[]  UngainTsProdOutMin=[]  UngainTsProdOutMax=[]  ClampingZeroOutDataTypeStr=Inherit: Inherit via back propagation  ClampingZeroOutMin=[]  ClampingZeroOutMax=[]  FilterDenConstantOutDataTypeStr=Inherit: Inherit via back propagation  FilterDenConstantOutMin=[]  FilterDenConstantOutMax=[]  PCopyOutDataTypeStr=Inherit: Inherit via back propagation  PCopyOutMin=[]  PCopyOutMax=[]  NCopyOutDataTypeStr=Inherit: Inherit via back propagation  NCopyOutMin=[]  NCopyOutMax=[]  IntegratorContinuousStateAttributes=''  IntegratorStateMustResolveToSignalObject=off  IntegratorRTWStateStorageClass=Auto  FilterContinuousStateAttributes=''  FilterStateMustResolveToSignalObject=off  FilterRTWStateStorageClass=Auto  ParallelPVariant=InternalParameters  IdealPVariant=Disabled  IVariant=InternalParameters  DVariant=InternalParameters  IntegratorVariant=Discrete  SatVariant=Disabled  AWVariant=Passthrough  PCopyVariant=Disabled  TRVariant=Disabled  FdbkBlocksVariant=Forward  IdealPFdbkVariant=Disabled  SatFdbkVariant=Disabled  DerivativeFilterVariant=ForwardEulerFilter  NVariant=InternalParameters  NCopyVariant=Disabled  FilterICVariant=InternalICsFilter  IntegratorICVariant=InternalICs  ExternalResetVariant=Disabled  TRSumVariant=Passthrough  SumFdbkVariant=Disabled  SumVariant=Sum_PID  TsampFilterVariant=InternalTs  TsampNgainVariant=Passthrough  TsampIntegralVariant=Disabled_SignalSpec  ExternalSaturationOutDataTypeStr=Inherit: Same as second input  DerivativeSourceVariant=ErrorSignal  PreIntVariant=InternalPreInt
  tag scope: Thrust=global, desired_pitch=global, desired_roll=global
  wires:
  [pd] -> Sum/2, Scope/1
  Sum/1 -> PID Controller/1
  [pe] -> Scope1/1, Sum1/2
  Sum1/1 -> PID Controller3/1
  Sum2/1 -> PID Controller2/1
  PID Controller/1 -> Gain2/1
  [pn] -> Scope2/1, Sum2/2
  Saturation/1 -> Scope3/1, [desired_pitch]
  PID Controller2/1 -> Gain1/1
  Gain1/1 -> Gain/1
  Gain/1 -> Saturation/1
  Add/1 -> Saturation2/1
  Constant1/1 -> Add/1
  Gain2/1 -> Add/2
  PID Controller3/1 -> Gain3/1
  Gain3/1 -> Saturation1/1
  Saturation1/1 -> [desired_roll]
  "Desired Altidude "/1 -> Sum/1
  Saturation2/1 -> [Thrust], Scope4/1
  Desired y postion/1 -> Sum1/1

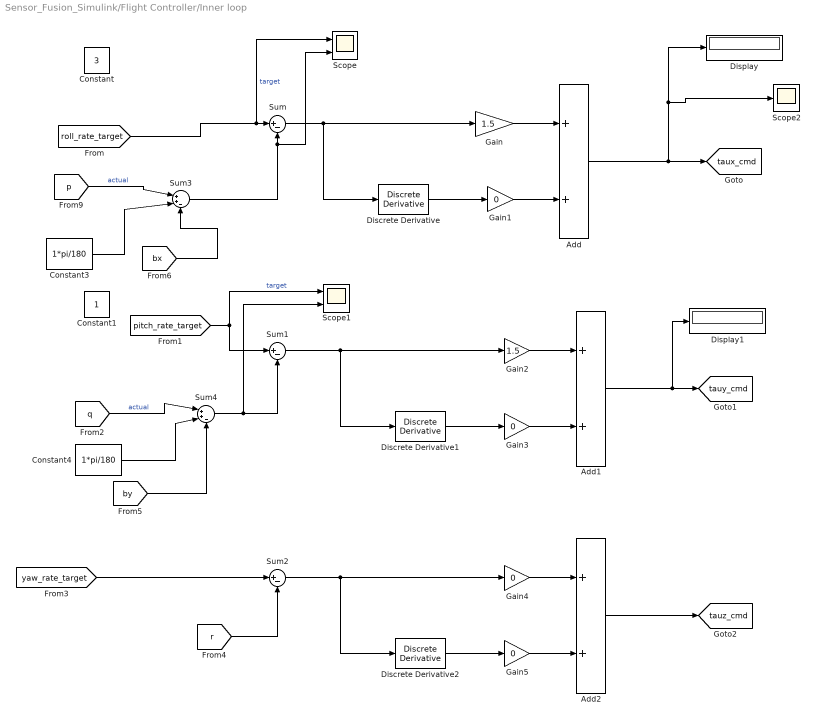
== system Sensor_Fusion_Simulink/Flight Controller/Inner loop ==
  Add : Sum
  Add1 : Sum
  Add2 : Sum
  Constant : Constant  Value=3
  Constant1 : Constant
  Constant3 : Constant  Value=1*pi/180
  Constant4 : Constant  Value=1*pi/180
  Discrete Derivative : simulink/Discrete/Discrete Derivative  gainval=1.0  ICPrevScaledInput=0.0  OutMin=[]  OutMax=[]  OutDataType=fixdt(1, 16)  OutScaling=2^-10  DoSatur=off
  Discrete Derivative1 : simulink/Discrete/Discrete Derivative  gainval=1.0  ICPrevScaledInput=0.0  OutMin=[]  OutMax=[]  OutDataType=fixdt(1, 16)  OutScaling=2^-10  DoSatur=off
  Discrete Derivative2 : simulink/Discrete/Discrete Derivative  gainval=1.0  ICPrevScaledInput=0.0  OutMin=[]  OutMax=[]  OutDataType=fixdt(1, 16)  OutScaling=2^-10  DoSatur=off
  Display : Display
  Display1 : Display
  Gain : Gain  Gain=1.5
  Gain{1,3..5} (4 alike) : Gain  Gain=0
  Gain2 : Gain  Gain=1.5
  Scope : Scope  NumInputPorts=2
      settings: ActiveDisplayYMinimum=-2.4043531105921616  ActiveDisplayYMaximum=7.2481570714437131  DataLoggingVariableName=ScopeData8
  Scope1 : Scope  NumInputPorts=2
      settings: ActiveDisplayYMinimum=-0.010746683981691024  ActiveDisplayYMaximum=0.026600766212361203  DataLoggingVariableName=ScopeData9
  Scope2 : Scope
      settings: ActiveDisplayYMinimum=-4.4078253508085865  ActiveDisplayYMaximum=10.932173658358906  DataLoggingVariableName=ScopeData10
  Sum : Sum  Inputs=|+-
  Sum1 : Sum  Inputs=|+-
  Sum2 : Sum  Inputs=|+-
  Sum3 : Sum  Inputs=|++-
  Sum4 : Sum  Inputs=|++-
  tag scope: taux_cmd=global, tauy_cmd=global, tauz_cmd=global
  wires:
  Sum/1 -> Discrete Derivative/1, Gain/1
  Gain1/1 -> Add/2
  Gain/1 -> Add/1
  Gain3/1 -> Add1/2
  Gain2/1 -> Add1/1
  Sum1/1 -> Discrete Derivative1/1, Gain2/1
  Discrete Derivative/1 -> Gain1/1
  Discrete Derivative1/1 -> Gain3/1
  Discrete Derivative2/1 -> Gain5/1
  Gain4/1 -> Add2/1
  Gain5/1 -> Add2/2
  [r] -> Sum2/2
  Sum2/1 -> Discrete Derivative2/1, Gain4/1
  Add/1 -> Scope2/1, Display/1, [taux_cmd]
  Add1/1 -> Display1/1, [tauy_cmd]
  Add2/1 -> [tauz_cmd]
  [roll_rate_target] -> Scope/1, Sum/1  "target"
  [pitch_rate_target] -> Scope1/1, Sum1/1  "target"
  Sum3/1 -> Scope/2, Sum/2
  [p] -> Sum3/1  "actual"
  Constant3/1 -> Sum3/2
  Sum4/1 -> Scope1/2, Sum1/2
  [q] -> Sum4/1  "actual"
  Constant4/1 -> Sum4/2
  [by] -> Sum4/3
  [bx] -> Sum3/3
  [yaw_rate_target] -> Sum2/1

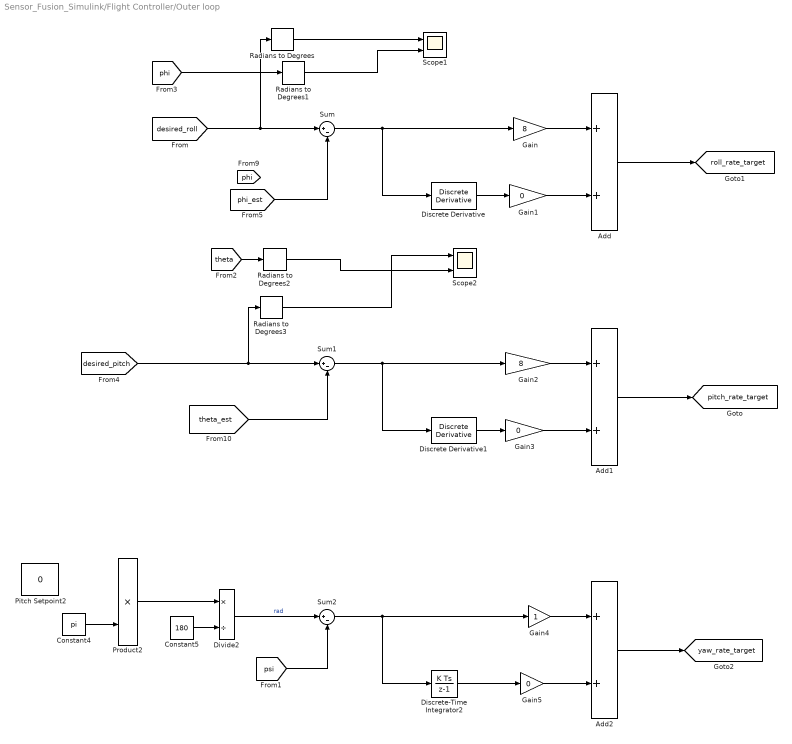
== system Sensor_Fusion_Simulink/Flight Controller/Outer loop ==
  Add : Sum
  Add1 : Sum
  Add2 : Sum
  Constant4 : Constant  Value=pi
  Constant5 : Constant  Value=180
  Discrete Derivative : simulink/Discrete/Discrete Derivative  gainval=1.0  ICPrevScaledInput=0.0  OutMin=[]  OutMax=[]  OutDataType=fixdt(1, 16)  OutScaling=2^-10  DoSatur=off
  Discrete Derivative1 : simulink/Discrete/Discrete Derivative  gainval=1.0  ICPrevScaledInput=0.0  OutMin=[]  OutMax=[]  OutDataType=fixdt(1, 16)  OutScaling=2^-10  DoSatur=off
  Discrete-Time Integrator2 : DiscreteIntegrator  SampleTime=-1  ICPrevOutput=DiscIntNeverNeededParam  ICPrevScaledInput=DiscIntNeverNeededParam
  Divide2 : Product  Inputs=*/
  Gain : Gain  Gain=8
  Gain1 : Gain  Gain=0
  Gain2 : Gain  Gain=8
  Gain3 : Gain  Gain=0
  Gain4 : Gain
  Gain5 : Gain  Gain=0
  Pitch Setpoint2 : Constant  Value=0
  Product2 : Product
  Radians to Degrees{,1..3} (4 alike) : simulink_extras/Transformations/Radians to Degrees
  Scope1 : Scope  NumInputPorts=2
      settings: ActiveDisplayYMinimum=-6.42420313917745  ActiveDisplayYMaximum=50.713800348797491  DataLoggingVariableName=ScopeData6
  Scope2 : Scope  NumInputPorts=2
      settings: ActiveDisplayYMinimum=-0.59119545198324364  ActiveDisplayYMaximum=0.95836540034532691  DataLoggingVariableName=ScopeData5
  Sum : Sum  Inputs=|+-
  Sum1 : Sum  Inputs=|+-
  Sum2 : Sum  Inputs=|+-
  tag scope: pitch_rate_target=global, roll_rate_target=global, yaw_rate_target=global
  wires:
  Sum/1 -> Discrete Derivative/1, Gain/1
  Gain3/1 -> Add1/2
  Gain1/1 -> Add/2
  Gain2/1 -> Add1/1
  Gain4/1 -> Add2/1
  Divide2/1 -> Sum2/1  "rad"
  Gain/1 -> Add/1
  Gain5/1 -> Add2/2
  Constant5/1 -> Divide2/2
  Sum2/1 -> Discrete-Time Integrator2/1, Gain4/1
  [psi] -> Sum2/2
  Constant4/1 -> Product2/2
  Product2/1 -> Divide2/1
  [theta_est] -> Sum1/2
  Add2/1 -> [yaw_rate_target]
  Discrete Derivative/1 -> Gain1/1
  Discrete Derivative1/1 -> Gain3/1
  Discrete-Time Integrator2/1 -> Gain5/1
  [theta] -> Radians to Degrees2/1
  [phi] -> Radians to Degrees1/1
  Sum1/1 -> Discrete Derivative1/1, Gain2/1
  Add/1 -> [roll_rate_target]
  Add1/1 -> [pitch_rate_target]
  Radians to Degrees/1 -> Scope1/1
  Radians to Degrees1/1 -> Scope1/2
  Radians to Degrees2/1 -> Scope2/2
  Radians to Degrees3/1 -> Scope2/1
  [desired_pitch] -> Radians to Degrees3/1, Sum1/1
  [desired_roll] -> Radians to Degrees/1, Sum/1
  [phi_est] -> Sum/2

== matlab function Sensor_Fusion_Simulink/Translational Kinematics and Dynamics/Translational Dynamics in Body Frame ==
  data: phi input; u_dot output; theta input; unused input; u input; v input; w input; T input; p input; q input; r input; v_dot output; w_dot output
function [u_dot, v_dot, w_dot] = fcn(phi, theta, ~, u, v, w, T, p, q, r)
m  = 1.2; 
g  = 9.81;
cd = 0.3;


ax = -(cd/m) * u;
ay = -(cd/m) * v;
az = -T / m;


u_dot = (r*v - q*w) + ax - g * sin(theta);
v_dot = (p*w - r*u) + ay + g * sin(phi) * cos(theta);
w_dot = (q*u - p*v) + az + g * cos(phi) * cos(theta);
end

== matlab function Sensor_Fusion_Simulink/EKF/Working on now ==
  settings: updateMethod=DISCRETE
  data: p input; q input; r input; ax input; ay input; az input; x_est output; P_out output; uk output; phi output; theta output; a_error output; a_magnitude output
function [x_est, P_out, uk, phi, theta, a_error, a_magnitude] = fcn(p, q, r, ax, ay, az)
    dt = 0.002;
    
    % Initialize persistent state estimates and covariance
    persistent x P Qd_est R_est;
    if isempty(x)
        x = [0; 0.0; 0.0; 0.0]; % Initial guess [phi; theta; bx; by]
        P = 0.001 * diag([0.01, 0.01, 0.01, 0.01]);       
        Qc_est = diag([1e-5, 1e-5, 1e-6, 1e-6]);
        Qd_est = Qc_est * dt;
        R_est = 0.02 * diag([1, 1]);
    end
    
    phi = x(1);
    theta = x(2);
    bx = x(3);
    by = x(4);
    
    c = [1 0 0 0;
         0 1 0 0]; 
    Ck = c;
    % 1. Time Update (Prediction Step using Gyroscope data)
    x = x + dt * [(p - bx) + (q - by)*sin(phi)*tan(theta) + r*cos(phi)*tan(theta);
                  (q - by)*cos(phi) - r*sin(phi);
                  0;
                  0];
    % Define Jacobian Matrix Ak
    Ak = eye(4) + dt * [ ...
        (q - by)*(cos(x(1))*tan(x(2))) - r*sin(x(1))*tan(x(2)), (q - by)*sin(x(1))*(1/cos(x(2))^2) + r*cos(x(1))*(1/cos(x(2))^2), -1, -sin(x(1))*tan(x(2)); 
        -q*sin(x(1)) + by*sin(x(1)) - r*cos(x(1)),                    0,                                                         0, -cos(x(1)); 
        0,                                                        0,                                                         0,  0; 
        0,                                                        0,                                                         0,  0];
    
    P = Ak * P * Ak' + Qd_est;
    
    % 2. Measurement Update with Acceleration Gating
    a_magnitude = sqrt(ax^2 + ay^2 + az^2);
    % Raw accelerometer angle measurements
    uk = [atan2(ay, az);
          atan2(-ax, sqrt(ay^2 + az^2))];
      
    a_error = abs(a_magnitude - 9.81);
    
    % Set R_current first so wk uses the correct inflated noise
    if a_error > 0.2
        R_current = R_est*1;
    else
        R_current = R_est;       
    end
  
    wk = P * Ck' / (Ck * P * Ck' + R_current); 
    % 
    % if a_error < 0.1
    %     wk(3:0) = 0;
    %     wk(4:0) = 0;
    % end
    % If acceleration error exceeds threshold, freeze bias estimation 
   
    y_inno = uk - c * x;
    x = x + wk * y_inno;
    
    x_est = x;
    % Compute error covariance matrices
    P = (eye(4) - wk * Ck) * P;
    P_out = P;
end

== matlab function Sensor_Fusion_Simulink/Translational Kinematics and Dynamics/MATLAB Function3 ==
  data: u_dot input; v_dot input; w_dot input; u input; v input; w input; p input; q input; r input; phi input; a_imu output; theta input
function a_imu = fcn(u_dot, v_dot, w_dot, u, v, w, p, q, r, phi, theta)

    g = 9.81;
    
    
    v_dot_vec = [u_dot; v_dot; w_dot];
    
   
    coriolis_vec = [q*w - r*v;
                    r*u - p*w;
                    p*v - q*u];
                    
   
    g_body_vec = [ -g * sin(theta);
                    g * sin(phi) * cos(theta);
                    g * cos(phi) * cos(theta) ];
                    
   
    a_imu = v_dot_vec + coriolis_vec + g_body_vec;

end

== matlab function Sensor_Fusion_Simulink/Rotational Kinematics and Dynamics/Rotational Dynamics ==
  data: p input; p_dot output; q input; r input; q_dot output; r_dot output; rotor1 input; rotor2 input; rotor3 input; rotor4 input
function [p_dot, q_dot, r_dot] = fcn(p, q, r, rotor1, rotor2, rotor3, rotor4)

rho = 1.225;
CQ = 0.012;
CT = 0.11;
L = 0.225;
g = 9.81;
%d = 0;
D = 0.3;
%Mass Moment of Inertia of the drone
jx = 0.015;
jy = 0.015;
jz = 0.028;

k = sqrt(2)/2;
%Mixing Matrix
M = ((rho*D^4)/(4*(pi^2)))*[  CT         CT       CT       CT;
                          -CQ*D*L*k -CQ*D*L*k CQ*D*L*k CQ*D*L*k;
                          CQ*D*L*k -CQ*D*L*k -CQ*D*L*k CQ*D*L*k;
                            CQ*D      -CQ*D    CQ*D     -CQ*D ];  
%Generating commands
command = M*[rotor1^2 rotor2^2 rotor3^2 rotor4^2]';

tau_b = [command(2) command(3) command(4)]';
%Mass Moment of inertial Matrix
J = [jx 0 0;
     0  jy 0;
     0  0  jz];

%Inversed Mass Moment of inertia matrix
J_inv = [1/jx 0 0;
        0  1/jy 0;
        0  0  1/jz];

omega_b = [p q r]';
%Calculating the body angular rates
omega_b_dot = J_inv * ((-cross(omega_b, (J * omega_b))) + tau_b);
p_dot = omega_b_dot(1);
q_dot = omega_b_dot(2);
r_dot = omega_b_dot(3);

== matlab function Sensor_Fusion_Simulink/Rotational Kinematics and Dynamics/Rotational Kinematics     ==
  data: p input; phi_dot output; q input; r input; theta_dot output; psi_dot output; phi input; theta input; psi input
function [phi_dot, theta_dot, psi_dot] = fcn(p, q, r, phi, theta, psi)

s_theta = [1 sin(phi)*tan(theta) cos(phi)*tan(theta);
           0       cos(phi)         -sin(phi);
           0        (sin(phi)/cos(theta))    (cos(phi)/cos(theta))];

euler_rate = s_theta * [p q r]';

phi_dot = euler_rate(1);
theta_dot = euler_rate(2);
psi_dot = euler_rate(3);

== matlab function Sensor_Fusion_Simulink/Translational Kinematics and Dynamics/Translational Dynamics in Global Frame ==
  data: phi input; vi_dot output; theta input; psi input; vi_n input; vi_e input; vi_d input; T input; constant output; constant2 output
function [vi_dot, constant, constant2] = fcn(phi, theta, psi, vi_n, vi_e, vi_d, T)
m  = 1.2; 
g  = 9.81;
cd = 0.3;

D = [cd 0 0;
     0   cd 0;
     0   0    0];

e3 = [0; 0; 1];
vi = [vi_n; vi_e; vi_d];

Rb_i = [cos(theta)*cos(psi)  sin(phi)*sin(theta)*cos(psi)-cos(phi)*sin(psi)  cos(phi)*sin(theta)*cos(psi)+sin(phi)*sin(psi);
        cos(theta)*sin(psi)  sin(phi)*sin(theta)*sin(psi)+cos(phi)*cos(psi)  cos(phi)*sin(theta)*sin(psi)-sin(phi)*cos(psi);
       -sin(theta)           sin(phi)*cos(theta)                             cos(phi)*cos(theta)];
Ri_b = Rb_i';

% Correct: Rb_i transforms thrust (body e3) to inertial, while Rb_i' rotates vi to body for drag
vi_dot = g*e3 - Rb_i*D*Ri_b*vi - (T/m)*Rb_i*e3;
constant =g*e3 - (T/m)*Rb_i*e3;
constant2 = Rb_i*D*Ri_b*vi;
end

== matlab function Sensor_Fusion_Simulink/Flight Controller/Motor Mixer ==
  data: taux_cmd input; rotor1 output; tauy_cmd input; tauz_cmd input; rotor2 output; rotor3 output; T input; rotor4 output
function [rotor1, rotor2, rotor3, rotor4] = fcn(taux_cmd, tauy_cmd, tauz_cmd, T)

rho = 1.225;
CQ = 0.012;
CT = 0.11;
L = 0.225;

D = 0.3; 
 
H = [T taux_cmd tauy_cmd tauz_cmd]';
k = sqrt(2)/2;


M = ((rho*D^4)/(4*pi^2))*[  CT         CT       CT       CT;
                        -CQ*D*L*k -CQ*D*L*k CQ*D*L*k CQ*D*L*k;
                        CQ*D*L*k -CQ*D*L*k -CQ*D*L*k CQ*D*L*k;
                          CQ*D      -CQ*D    CQ*D     -CQ*D ];  

rotors_square = M\H;

rotors_square_clamped = max(rotors_square, 0);


rotor1 = sqrt(rotors_square_clamped(1));
rotor2 = sqrt(rotors_square_clamped(2));
rotor3 = sqrt(rotors_square_clamped(3));
rotor4 = sqrt(rotors_square_clamped(4));

== matlab function Sensor_Fusion_Simulink/Flight Controller/Altitude Control/MATLAB Function ==
  data: u input; y output
function y = fcn(u)

y = u;
